simulink model "test_SimulinkMdl2_qLPVMPCbeta_UIO_testOL"  (R2019b)
settings: Solver=FixedStepAuto  StartTime=0.0  StopTime=400  FixedStep=DT  RelTol=1e-3
values from neighbouring files (symbols this model uses):
  beta = [-0.13962634015954636; -0.1361356816555577; -0.13264502315156904;          -0.12915436464758037; -0.12566370614359171; -0.12217304763960307;          -0.11868238913561441; -0.11519173063162574; -0.11170107212763709;          -0.10821041362364842; -0.10471975511965977; -0.10122909661567112;          -0.097738438111682452; -0.094247779607693788; -0.09075712110370511;          -0.087266462599716474;  ...(+3598 chars)    [MdlMFile.m]
  Cq = saveVarsMat.Cq    [MdlMFile.m]
  Ct = saveVarsMat.Ct    [MdlMFile.m]
  DT = 0.008    [LUTMFile.m]    (also in UIOLinestTr.m; exUIO_WECS.m; getFictInputMatricesOrd3M.m; initWorkspace.m)
  lambda = [0; 0.1; 0.2; 0.30000000000000004; 0.4; 0.5; 0.60000000000000009;            0.70000000000000007; 0.8; 0.9; 1; 1.1; 1.2000000000000002; 1.3;            1.4000000000000001; 1.5; 1.6; 1.7000000000000002; 1.8; 1.9000000000000001;            2; 2.1; 2.2; 2.3000000000000003; 2.4000000000000004; 2.5; 2.6;            2.7; 2.8000000000000003; 2.9000000000000004; 3; 3.1; 3.2; 3.3000000000000003;            ...(+1285 chars)    [MdlMFile.m]    (also in exLQR_hamiltonian.m = -10; koopmanKhalil.m = 1)
  Lin_points = 0.74811652133345019 0.78122947334555715 0.82586806925039735 0.88042797952230989 0.94564154658981237 1.06231329175348 1.1780905557148451 1.2402773842094346 1.254474305465946 1.2544764615597244 1.2544775037226534 1.2544778841663968 1.2544780221694662 1.2544779823335293 1.254477987181289 1.2544781738200332 1.254478189259095 1.2544780953600987 1.2544781548505395 1.2544783366942183 1.2544785605869417 1    [DD_test.sldd]    (also in LinPointsMFile.m = struct)
  rho = 1.2250    (= 1.225)    [ABqL_WT_est_matlab.m]    (also in MdlMFile.m; UIOLinestTr.m; getFictInputMatricesOrd3M.m; testTorqueFromomegaNonLin.m)
  sysEst = c2d(ss(F,[T*B,K],eye(nx),[zeros(size(T*B)),H]),DT,'zoh')    [exUIO_WECS.m]
  Vbar = rhoP(3)    [ABqL_WT_est_matlab.m]    (also in checkOPSimulink.m = Lin_points.V(index); createLinearModels.m = Lin.V(index); getFictInputMatricesOrd3M.m = wind - zetadot*rb - ytdot)
  wecs = 3.0    [DD_test.sldd]    (also in MdlMFile.m = struct)
undefined symbols (not defined in the file or in its folder): Rotor_Lambda
settings Model: ExtModeTrigMode=oneshot  ExtModeArmWhenConnect=off  Creator=Hazim Namik  LastModifiedBy=ditt_aj
settings DataIOCC: LimitDataPoints=on  SaveFormat=Array  ReturnWorkspaceOutputs=off
settings OptimizationCC: BlockReduction=off  BooleanDataType=off  LifeSpan=inf
settings DebuggingCC: SaveWithParameterizedLinksMsg=none  UnderspecifiedInitializationDetection=Classic  MergeDetectMultiDrivingBlocksExec=none  SignalResolutionControl=TryResolveAllWithWarning  SFUnexpectedBacktrackingDiag=warning  SFNoUnconditionalDefaultTransitionDiag=warning  SFExecutionAtInitializationDiag=none  ArithmeticOperatorsInVariantConditions=warning
settings HardwareCC: ProdBitPerPointer=32  ProdBitPerSizeT=32  ProdBitPerPtrDiffT=32  ProdLargestAtomicFloat=None  ProdIntDivRoundTo=Undefined  ProdEndianess=Unspecified  ProdWordSize=32  ProdHWDeviceType=32-bit Generic  TargetUnknown=on
settings ModelReferenceCC: PropagateSignalLabelsOutOfModel=off
settings SFSimCC: SimUseLocalCustomCode=off  CustomCodeUndefinedFunction=UseInterfaceOnly
settings RTWCC: RTWUseLocalCustomCode=off
settings CodeAppCC: StateflowObjectComments=on
settings GRTTargetCC: TargetLangStandard=C89/C90 (ANSI)  GeneratePreprocessorConditionals=Disable all
settings ConfigComp: CovMetricSettings=dw  CovHtmlReporting=on  CovSaveCumulativeToWorkspaceVar=on  CovSaveSingleToWorkspaceVar=on  CovExternalEMLEnable=off

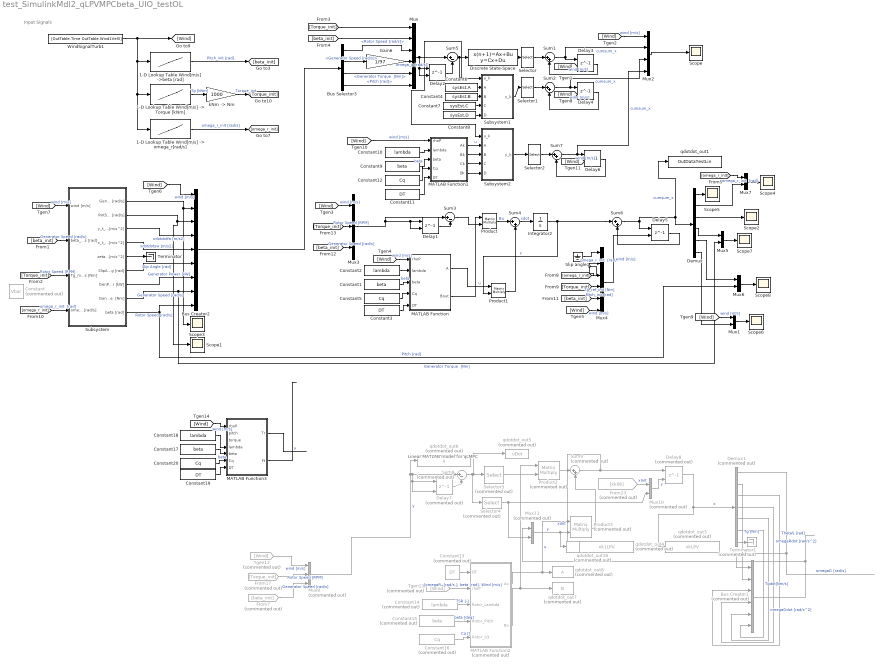
== system test_SimulinkMdl2_qLPVMPCbeta_UIO_testOL ==
  note: Input Signals
  note: Linear MATLAB model for qLMPC
  "1-D Lookup Table Wind[m/s] -> Torque [kNm]" : Lookup_n-D  NumberOfTableDimensions=1  BreakpointsForDimension1=Lin_points.V  BreakpointsForDimension2=Rotor_Lambda  Table=Lin_points.Torque  InternalRulePriority=Speed  RndMeth=Simplest  InputSameDT=on
  "1-D Lookup Table Wind[m/s] -> omega_r[rad/s]" : Lookup_n-D  NumberOfTableDimensions=1  BreakpointsForDimension1=Lin_points.V  BreakpointsForDimension2=Rotor_Lambda  Table=Lin_points.RSpeed  InternalRulePriority=Speed  RndMeth=Simplest  InputSameDT=on
  1-D Lookup Table Wind[m/s] ->beta [rad] : Lookup_n-D  NumberOfTableDimensions=1  BreakpointsForDimension1=Lin_points.V  BreakpointsForDimension2=Rotor_Lambda  Table=Lin_points.Pitch  InternalRulePriority=Speed  RndMeth=Simplest  InputSameDT=on
  Bus Creator1 : BusCreator  Commented=on  Inputs=6
  Bus Creator2 : BusCreator  Inputs=9
  Bus Selector3 : BusSelector  OutputSignals="Rotor Speed [rad/s],Generator Speed [rad/s],Generator Torque  [Nm],Pitch [rad]"
  Constant : Constant  Commented=on  Value=Vbar
  Constant1 : Constant  Value=beta
  Constant10 : Constant  Value=lambda
  Constant11 : Constant  Value=DT
  Constant12 : Constant  Value=Cq
  Constant13 : Constant  Commented=on  Value=DT
  Constant14 : Constant  Commented=on  Value=lambda
  Constant15 : Constant  Commented=on  Value=beta
  Constant16 : Constant  Commented=on  Value=Cq
  Constant17 : Constant  Value=beta
  Constant18 : Constant  Value=lambda
  Constant19 : Constant  Value=DT
  Constant2 : Constant  Value=lambda
  Constant20 : Constant  Value=Cq
  Constant3 : Constant  Value=DT
  Constant4 : Constant  Value=sysEst.B
  Constant5 : Constant  Value=Cq
  Constant6 : Constant  Value=sysEst.A
  Constant7 : Constant  Value=sysEst.C
  Constant8 : Constant  Value=sysEst.D
  Constant9 : Constant  Value=beta
  Delay{1..6} (6 alike) : Delay  DelayLength=1  InitialConditionSource=Input port  InitialCondition=0
      settings: InputPortMap=u0,p4
  Delay7 : Delay  Commented=on  DelayLength=1  InitialConditionSource=Input port  InitialCondition=[0, Lin_points.Torque(1)]
      settings: InputPortMap=u0,p4
  Delay8 : Delay  Commented=on  DelayLength=1  InitialConditionSource=Input port
      settings: InputPortMap=u0,p4
  Demux : Demux  Outputs=6
  Demux1 : Demux  Commented=on  Outputs=7
  Discrete State-Space : DiscreteStateSpace  A=sysEst.A  B=sysEst.B  C=sysEst.C  D=sysEst.D  SampleTime=DT
  From17 : From  Commented=on  GotoTag=Torque_init
      settings: CloseFcn=tagdialog Close
  From23 : From  Commented=on  GotoTag=xk06
      settings: CloseFcn=tagdialog Close
  From7 : From  Commented=on  GotoTag=beta_init
      settings: CloseFcn=tagdialog Close
  Gain6 : Gain  Gain=1/97
  Integrator2 : Integrator
  MATLAB Function : MATLAB Function  TreatAsAtomicUnit=on
  MATLAB Function1 : MATLAB Function  TreatAsAtomicUnit=on
  MATLAB Function2 : MATLAB Function  Commented=on  TreatAsAtomicUnit=on
  MATLAB Function3 : MATLAB Function  TreatAsAtomicUnit=on
  Mux : Mux  Inputs=6
  Mux{1,5..7} (4 alike) : Mux  Inputs=2
  Mux10 : Mux  Commented=on  Inputs=2
  Mux11 : Mux  Commented=on  Inputs=2
  Mux2 : Mux
  Mux3 : Mux  Inputs=3
  Mux4 : Mux  Inputs=6
  Mux8 : Mux  Commented=on  Inputs=3
  Product : Product  Multiplication=Matrix(*)
  Product1 : Product  Multiplication=Matrix(*)
  Product2 : Product  Commented=on  Multiplication=Matrix(*)  RndMeth=Zero
  Product3 : Product  Commented=on  Multiplication=Matrix(*)  RndMeth=Zero
  Scope{,1..8} (9 alike) : Scope
  Selector : Selector  InputPortWidth=size(sysEst.C,1)  IndexOptions=Index vector (dialog)  Indices=size(sysEst.C,1)  OutputSizes=1
  Selector1 : Selector  InputPortWidth=size(sysEst.C,1)  IndexOptions=Index vector (dialog)  Indices=size(sysEst.C,1)  OutputSizes=1
  Selector2 : Selector  InputPortWidth=size(sysEst.C,1)  IndexOptions=Index vector (dialog)  Indices=size(sysEst.C,1)  OutputSizes=1
  Selector3 : Selector  Commented=on  InputPortWidth=3  IndexOptions=Index vector (dialog)  Indices=[2 3]  OutputSizes=1
  Selector4 : Selector  Commented=on  InputPortWidth=3  IndexOptions=Index vector (dialog)  Indices=1  OutputSizes=1
  Slip angle1 : Ground
  Subsystem : Subsystem
  Subsystem1 : Subsystem
  Subsystem2 : Subsystem
  Sum{1..2,4,6..7} (5 alike) : Sum  Inputs=|++
  Sum3 : Sum  Inputs=|+-
  Sum5 : Sum  Inputs=|+-
  Sum8 : Sum  Commented=on  Inputs=|+-
  Sum9 : Sum  Commented=on  Inputs=|++
  Terminator : Terminator
  Terminator1 : Terminator  Commented=on
  Tgen12 : From  Commented=on  GotoTag=Wind
      settings: CloseFcn=tagdialog Close
  Tgen13 : From  Commented=on  GotoTag=Wind
      settings: CloseFcn=tagdialog Close
  WindSignalTurb1 : FromWorkspace  VariableName=[OutTable.Time OutTable.Wind1VelX]  SampleTime=DT  OutputAfterFinalValue=Holding final value
  "kNm -> Nm" : Gain  Gain=1000
  qdotdot_out1 : ToWorkspace  VariableName=OutDataTestLin  SampleTime=-1
  qdotdot_out19 : ToWorkspace  Commented=on  VariableName=xkLPV1  SampleTime=-1
  qdotdot_out3 : ToWorkspace  Commented=on  VariableName=xkLPV  SampleTime=-1
  qdotdot_out4 : ToWorkspace  Commented=on  VariableName=xk1LPV  SampleTime=-1
  qdotdot_out5 : ToWorkspace  Commented=on  VariableName=uDot  SampleTime=-1
  qdotdot_out6 : ToWorkspace  Commented=on  VariableName=u  SampleTime=-1
  qdotdot_out7 : ToWorkspace  Commented=on  VariableName=B  SampleTime=-1
  qdotdot_out8 : ToWorkspace  Commented=on  VariableName=A  SampleTime=-1
  wires:
  Subsystem/7(GenPwr [kW]) -> Bus Creator2/7  "Generator Power [kW]"
  WindSignalTurb1/1 -> [Wind], "1-D Lookup Table Wind[m/s] -> omega_r[rad/s]"/1, "1-D Lookup Table Wind[m/s] -> Torque [kNm]"/1, 1-D Lookup Table Wind[m/s] ->beta [rad]/1
  Subsystem/3(y_t_dotdot [m/s^2]) -> Bus Creator2/4  "xdotdotfa [m/s2]"
  Subsystem/6(SlipAng [rad]) -> Bus Creator2/6  "Slip Angle [rad]"
  "kNm -> Nm"/1 -> [Torque_init]  "Torque_init"
  Bus Creator2/1 -> Bus Selector3/1
  Subsystem/2(" RotSpeed [rad/s]") -> Scope1/1, Bus Creator2/3  "Rotor Speed [rad/s]"
  [Torque_init] -> Subsystem/3(Tg_meas [Nm])  "Rotor Speed [RPM]"
  [Wind] -> Bus Creator2/1  "wind [m/s]"
  Subsystem/4(x_t_dotdot [m/s^2]) -> Bus Creator2/5  "xdotdotsw [m/s2]"
  Subsystem/1("GenSpeed [rad/s] ") -> Scope3/1, Bus Creator2/2  "Generator Speed [rad/s]"
  "1-D Lookup Table Wind[m/s] -> omega_r[rad/s]"/1 -> [omega_r_init]  "omega_r_init [rad/s]"
  [Wind] -> Subsystem/1(wind [m/s])  "wind [m/s]"
  1-D Lookup Table Wind[m/s] ->beta [rad]/1 -> [beta_init]  "Pitch_init [rad]"
  "1-D Lookup Table Wind[m/s] -> Torque [kNm]"/1 -> "kNm -> Nm"/1  "Tg [kNm]"
  Subsystem/9(beta [rad]) -> Bus Creator2/9, Mux6/2  "Pitch [rad]"
  Subsystem/8("GenTorque  [Nm]  ") -> Mux5/2, Bus Creator2/8  "Generator Torque  [Nm]"
  Subsystem/5(zeta_dotdot [m/s^2]) -> Terminator/1
  [beta_init] -> Subsystem/2(beta_meas [rad])  "Generator Speed [rad/s]"
  [omega_r_init] -> Subsystem/4(omega_init [rad/s])  "omega_r_init  [rad]"
  Bus Selector3/1 -> Mux/3  "<Rotor Speed [rad/s]>"
  Bus Selector3/2 -> Gain6/1  "<Generator Speed [rad/s]>"
  Discrete State-Space/1 -> Selector/1
  Mux2/1 -> Scope/1
  [Wind] -> Mux2/1  "wind [m/s]"
  Subsystem1/1(y_k) -> Selector1/1
  [Torque_init] -> Mux/1
  [beta_init] -> Mux/2
  Bus Selector3/4 -> Mux/6  "<Pitch [rad]>"
  Bus Selector3/3 -> Mux/5  "<Generator Torque  [Nm]>"
  Gain6/1 -> Mux/4  "omega_g [rad/s]]"
  Constant2/1 -> MATLAB Function/2(lambda)
  Constant5/1 -> MATLAB Function/4(Cq)
  Constant1/1 -> MATLAB Function/3(beta)  "beta"
  Product/1 -> Sum4/1  "Bu"
  Integrator2/1 -> Sum6/1, Product1/2  "x"
  Sum4/1 -> Integrator2/1  "xdot"
  MATLAB Function/1(A) -> Product1/1  "u"
  MATLAB Function/2(Bout) -> Product/1
  Product1/1 -> Sum4/2
  Demux/3 -> Scope2/1
  Slip angle1/1 -> Mux4/1
  [beta_init] -> Mux4/5  "Pitch_init [rad]"
  [omega_r_init] -> Mux4/2, Mux4/3  "omega_r_init  [rad]"
  [Torque_init] -> Mux4/4  "Tg_ref_init [Nm]"
  Demux/1 -> Scope5/1
  Demux/4 -> Mux5/1
  Mux5/1 -> Scope7/1
  Mux6/1 -> Scope8/1
  Demux/5 -> Mux6/1
  [Wind] -> Mux3/1  "wind [m/s]"
  [beta_init] -> Mux3/3  "Generator Speed [rad/s]"
  [Torque_init] -> Mux3/2  "Rotor Speed [RPM]"
  Mux7/1 -> Scope4/1
  Mux3/1 -> Delay1/2, Delay1/1, Sum3/1
  Delay1/1 -> Sum3/2
  Sum3/1 -> Product/2
  [Wind] -> MATLAB Function/1(rhoP)  "wind [m/s]"
  Constant3/1 -> MATLAB Function/5(DT)
  [Wind] -> Mux4/6  "wind [m/s]"
  Sum1/1 -> Delay3/1, Mux2/2  "cumsum_x"
  Delay3/1 -> Sum1/2
  [Wind] -> Delay3/2  "wind [m/s]"
  Selector/1 -> Sum1/1
  Sum2/1 -> Mux2/3, Delay4/1  "cumsum_x"
  [Wind] -> Delay4/2  "wind [m/s]"
  Delay4/1 -> Sum2/2
  Selector1/1 -> Sum2/1
  Mux/1 -> Delay2/1, Delay2/2, Sum5/1
  Delay2/1 -> Sum5/2
  Sum5/1 -> Subsystem2/1(u_k), Subsystem1/1(u_k), Discrete State-Space/1
  Mux4/1 -> Delay5/2  "wind [m/s]"
  Delay5/1 -> Sum6/2
  Sum6/1 -> qdotdot_out1/1, Demux/1, Delay5/1  "cumsum_x"
  Mux1/1 -> Scope6/1
  Demux/6 -> Mux1/2
  [Wind] -> Mux1/1  "wind [m/s]"
  Constant6/1 -> Subsystem1/2(A)
  Constant4/1 -> Subsystem1/3(B)
  Constant7/1 -> Subsystem1/4(C)
  Constant8/1 -> Subsystem1/5(D)
  [Wind] -> MATLAB Function1/1(rhoP)  "wind [m/s]"
  Constant10/1 -> MATLAB Function1/2(lambda)
  Constant12/1 -> MATLAB Function1/4(Cq)
  Constant9/1 -> MATLAB Function1/3(beta)  "beta"
  Constant11/1 -> MATLAB Function1/5(DT)
  MATLAB Function1/1(Ak) -> Subsystem2/2(A)  "u"
  MATLAB Function1/2(Bk) -> Subsystem2/3(B)
  MATLAB Function1/3(Ck) -> Subsystem2/4(C)
  MATLAB Function1/4(Dk) -> Subsystem2/5(D)
  Selector2/1 -> Sum7/1
  [Wind] -> Delay6/2  "wind [m/s]"
  Delay6/1 -> Sum7/2
  Sum7/1 -> Mux2/4, Delay6/1  "cumsum_x"
  Subsystem2/1(y_k) -> Selector2/1
  Demux/2 -> Mux7/2
  [omega_r_init] -> Mux7/1  "omega_r_init  [rad]"
  Mux8/1 -> qdotdot_out6/1, Delay7/1, Delay7/2, Sum8/1  "y"
  Selector4/1 -> Mux11/2, Mux10/2
  Selector3/1 -> Product2/2
  MATLAB Function2/2(Bv) -> qdotdot_out7/1, Product2/1
  Demux1/2 -> Bus Creator1/2  "Tg [Nm]"
  Sum9/1 -> Delay8/1, qdotdot_out4/1  "xdot"
  MATLAB Function2/1(Av) -> Product3/1, qdotdot_out8/1  "u"
  Sum8/1 -> Selector4/1, Selector3/1, qdotdot_out5/1
  Delay8/1 -> Demux1/1, qdotdot_out3/1  "x"
  Tgen13/1 -> MATLAB Function2/2(rhoP)  "[omegaR  [rad/s,], beta [rad], Wind [m/s]"
  Mux11/1 -> qdotdot_out19/1, Product3/2  "y"
  Bus Creator1/1 -> Mux11/1
  Demux1/5 -> Bus Creator1/5  "omegaGdot [rad/s^2]"
  Demux1/4 -> Bus Creator1/4  "omegaRdot [rad/s^2]"
  Demux1/3 -> Bus Creator1/3  "ThetaS [rad]"
  Demux1/7 -> Terminator1/1
  Delay7/1 -> Sum8/2
  Constant15/1 -> MATLAB Function2/4(Rotor_Pitch)  "beta [deg]"
  Demux1/1 -> Bus Creator1/1  "omegaG [rad/s]"
  Demux1/6 -> Bus Creator1/6  "Tgdot[Nm/s]"
  Mux10/1 -> Delay8/2  "y"
  Constant13/1 -> MATLAB Function2/1(DT)
  Product2/1 -> Sum9/1
  Constant16/1 -> MATLAB Function2/5(Rotor_cQ)  "Cq []"
  Constant14/1 -> MATLAB Function2/3(Rotor_Lambda)  "TSR [-]"
  From23/1 -> Mux10/1  "xInit"
  Product3/1 -> Sum9/2
  Tgen12/1 -> Mux8/1  "wind [m/s]"
  From17/1 -> Mux8/2  "Rotor Speed [RPM]"
  From7/1 -> Mux8/3  "Generator Speed [rad/s]"
  Constant19/1 -> MATLAB Function3/7(DT)
  MATLAB Function3/2(Ft) -> ?
  Constant17/1 -> MATLAB Function3/5(beta)  "beta"
  MATLAB Function3/1(Tr) -> ?  "u"
  Constant20/1 -> MATLAB Function3/6(Cq)
  [Wind] -> MATLAB Function3/1(rhoP)  "wind [m/s]"
  Constant18/1 -> MATLAB Function3/4(lambda)

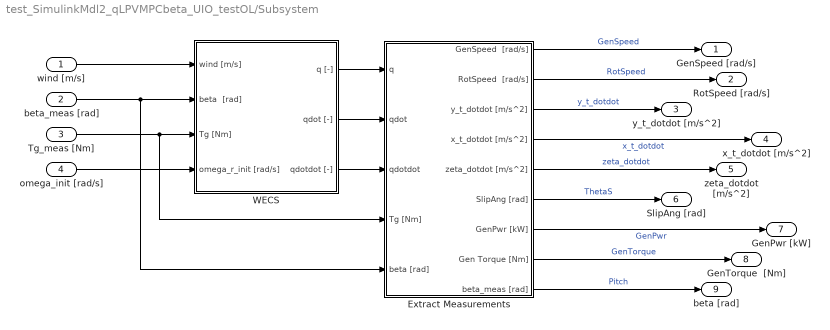
== system test_SimulinkMdl2_qLPVMPCbeta_UIO_testOL/Subsystem ==
  wind [m/s] : Inport
  beta_meas [rad] : Inport  Port=2
  Tg_meas [Nm] : Inport  Port=3
  omega_init [rad/s] : Inport  Port=4
  Extract Measurements : Subsystem
  WECS : Subsystem
  "GenSpeed [rad/s] " : Outport  VectorParamsAs1DForOutWhenUnconnected=off
  " RotSpeed [rad/s]" : Outport  Port=2  VectorParamsAs1DForOutWhenUnconnected=off
  y_t_dotdot [m/s^2] : Outport  Port=3  VectorParamsAs1DForOutWhenUnconnected=off
  x_t_dotdot [m/s^2] : Outport  Port=4  VectorParamsAs1DForOutWhenUnconnected=off
  zeta_dotdot [m/s^2] : Outport  Port=5  VectorParamsAs1DForOutWhenUnconnected=off
  SlipAng [rad] : Outport  Port=6  VectorParamsAs1DForOutWhenUnconnected=off
  GenPwr [kW] : Outport  Port=7  VectorParamsAs1DForOutWhenUnconnected=off
  "GenTorque  [Nm]  " : Outport  Port=8  VectorParamsAs1DForOutWhenUnconnected=off
  beta [rad] : Outport  Port=9  VectorParamsAs1DForOutWhenUnconnected=off
  wires:
  omega_init [rad/s]/1 -> WECS/4(omega_r_init [rad/s])
  beta_meas [rad]/1 -> WECS/2(beta  [rad]), Extract Measurements/5(beta [rad])
  Extract Measurements/3(y_t_dotdot [m/s^2]) -> y_t_dotdot [m/s^2]/1  "y_t_dotdot"
  wind [m/s]/1 -> WECS/1(wind [m/s])
  Extract Measurements/8("Gen Torque [Nm]  ") -> "GenTorque  [Nm]  "/1  "GenTorque"
  Extract Measurements/4(x_t_dotdot [m/s^2]) -> x_t_dotdot [m/s^2]/1  "x_t_dotdot"
  WECS/1(q [-]) -> Extract Measurements/1(q)
  Tg_meas [Nm]/1 -> WECS/3(Tg [Nm]), Extract Measurements/4(Tg [Nm])
  Extract Measurements/5(zeta_dotdot [m/s^2]) -> zeta_dotdot [m/s^2]/1  "zeta_dotdot"
  Extract Measurements/2(RotSpeed  [rad/s]) -> " RotSpeed [rad/s]"/1  "RotSpeed"
  WECS/2(qdot [-]) -> Extract Measurements/2(qdot)
  Extract Measurements/1(GenSpeed  [rad/s]) -> "GenSpeed [rad/s] "/1  "GenSpeed"
  Extract Measurements/9(beta_meas [rad]) -> beta [rad]/1  "Pitch"
  Extract Measurements/6(SlipAng [rad]) -> SlipAng [rad]/1  "ThetaS"
  WECS/3(qdotdot [-]) -> Extract Measurements/3(qdotdot)
  Extract Measurements/7(GenPwr [kW]) -> GenPwr [kW]/1  "GenPwr"

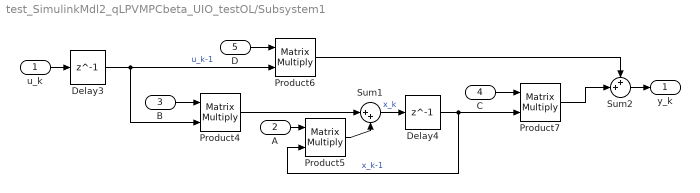
== system test_SimulinkMdl2_qLPVMPCbeta_UIO_testOL/Subsystem1 ==
  u_k : Inport
  A : Inport  Port=2
  B : Inport  Port=3
  C : Inport  Port=4
  D : Inport  Port=5
  Delay3 : Delay  DelayLength=1
  Delay4 : Delay  DelayLength=1
  Product{4..7} (4 alike) : Product  Multiplication=Matrix(*)
  Sum1 : Sum  Inputs=|++
  Sum2 : Sum  Inputs=++|
  y_k : Outport
  wires:
  Delay4/1 -> Product5/2, Product7/2  "x_k-1"
  u_k/1 -> Delay3/1
  Product7/1 -> Sum2/2
  C/1 -> Product7/1
  Product6/1 -> Sum2/1
  Delay3/1 -> Product4/2, Product6/2  "u_k-1"
  Product5/1 -> Sum1/2
  D/1 -> Product6/1
  Product4/1 -> Sum1/1
  A/1 -> Product5/1
  Sum1/1 -> Delay4/1  "x_k"
  B/1 -> Product4/1
  Sum2/1 -> y_k/1

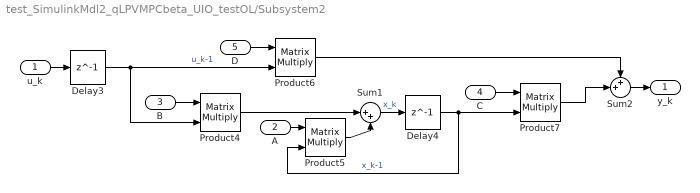
== system test_SimulinkMdl2_qLPVMPCbeta_UIO_testOL/Subsystem2 ==
  u_k : Inport
  A : Inport  Port=2
  B : Inport  Port=3
  C : Inport  Port=4
  D : Inport  Port=5
  Delay3 : Delay  DelayLength=1
  Delay4 : Delay  DelayLength=1
  Product{4..7} (4 alike) : Product  Multiplication=Matrix(*)
  Sum1 : Sum  Inputs=|++
  Sum2 : Sum  Inputs=++|
  y_k : Outport
  wires:
  Delay4/1 -> Product5/2, Product7/2  "x_k-1"
  u_k/1 -> Delay3/1
  Product7/1 -> Sum2/2
  C/1 -> Product7/1
  Product6/1 -> Sum2/1
  Delay3/1 -> Product4/2, Product6/2  "u_k-1"
  Product5/1 -> Sum1/2
  D/1 -> Product6/1
  Product4/1 -> Sum1/1
  A/1 -> Product5/1
  Sum1/1 -> Delay4/1  "x_k"
  B/1 -> Product4/1
  Sum2/1 -> y_k/1

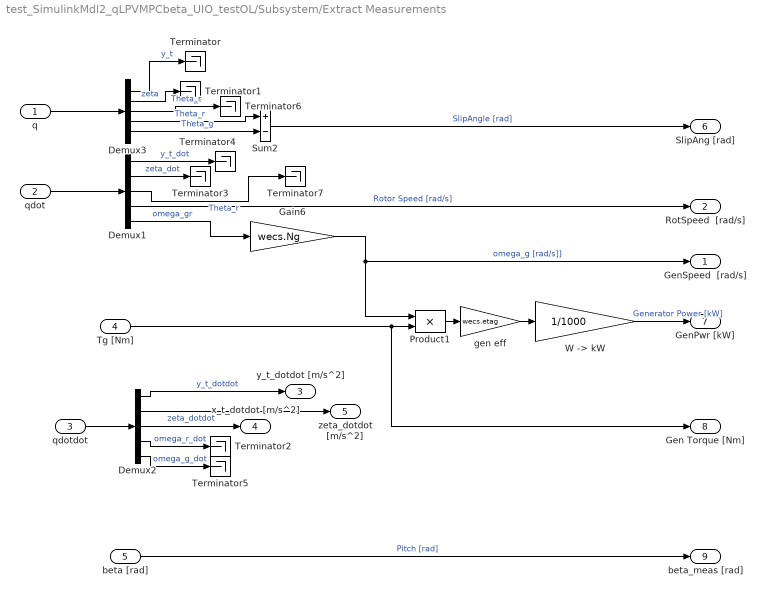
== system test_SimulinkMdl2_qLPVMPCbeta_UIO_testOL/Subsystem/Extract Measurements ==
  q : Inport
  qdot : Inport  Port=2
  qdotdot : Inport  Port=3
  Tg [Nm] : Inport  Port=4
  beta [rad] : Inport  Port=5
  Demux1 : Demux  Outputs=5
  Demux2 : Demux  Outputs=5
  Demux3 : Demux  Outputs=5
  Gain6 : Gain  Gain=wecs.Ng
  Product1 : Product  RndMeth=Zero
  Sum2 : Sum  Inputs=+-
  Terminator{,1..7} (8 alike) : Terminator
  "W -> kW" : Gain  Gain=1/1000
  gen eff : Gain  Gain=wecs.etag
  GenSpeed  [rad/s] : Outport  VectorParamsAs1DForOutWhenUnconnected=off
  RotSpeed  [rad/s] : Outport  Port=2  VectorParamsAs1DForOutWhenUnconnected=off
  y_t_dotdot [m/s^2] : Outport  Port=3  VectorParamsAs1DForOutWhenUnconnected=off
  x_t_dotdot [m/s^2] : Outport  Port=4  VectorParamsAs1DForOutWhenUnconnected=off
  zeta_dotdot [m/s^2] : Outport  Port=5  VectorParamsAs1DForOutWhenUnconnected=off
  SlipAng [rad] : Outport  Port=6  VectorParamsAs1DForOutWhenUnconnected=off
  GenPwr [kW] : Outport  Port=7  VectorParamsAs1DForOutWhenUnconnected=off
  "Gen Torque [Nm]  " : Outport  Port=8  VectorParamsAs1DForOutWhenUnconnected=off
  beta_meas [rad] : Outport  Port=9  VectorParamsAs1DForOutWhenUnconnected=off
  wires:
  Demux1/2 -> Terminator3/1  "zeta_dot"
  Demux2/1 -> y_t_dotdot [m/s^2]/1  "y_t_dotdot"
  Gain6/1 -> GenSpeed  [rad/s]/1, Product1/1  "omega_g [rad/s]]"
  Demux1/1 -> Terminator4/1  "y_t_dot"
  qdot/1 -> Demux1/1
  Demux3/4 -> Sum2/1  "Theta_r"
  Demux3/5 -> Sum2/2  "Theta_g"
  Demux2/5 -> Terminator5/1  "omega_g_dot"
  Tg [Nm]/1 -> "Gen Torque [Nm]  "/1, Product1/2
  Demux2/4 -> Terminator2/1  "omega_r_dot"
  Sum2/1 -> SlipAng [rad]/1  "SlipAngle [rad]"
  Demux1/5 -> Gain6/1  "omega_gr"
  Product1/1 -> gen eff/1
  Demux3/2 -> Terminator1/1  "zeta"
  Demux2/2 -> zeta_dotdot [m/s^2]/1  "zeta_dotdot"
  Demux3/1 -> Terminator/1  "y_t"
  gen eff/1 -> "W -> kW"/1
  "W -> kW"/1 -> GenPwr [kW]/1  "Generator Power [kW]"
  q/1 -> Demux3/1
  qdotdot/1 -> Demux2/1
  Demux1/4 -> RotSpeed  [rad/s]/1  "Rotor Speed [rad/s]"
  beta [rad]/1 -> beta_meas [rad]/1  "Pitch [rad]"
  Demux2/3 -> x_t_dotdot [m/s^2]/1
  Demux3/3 -> Terminator6/1  "Theta_r"
  Demux1/3 -> Terminator7/1  "Theta_r"

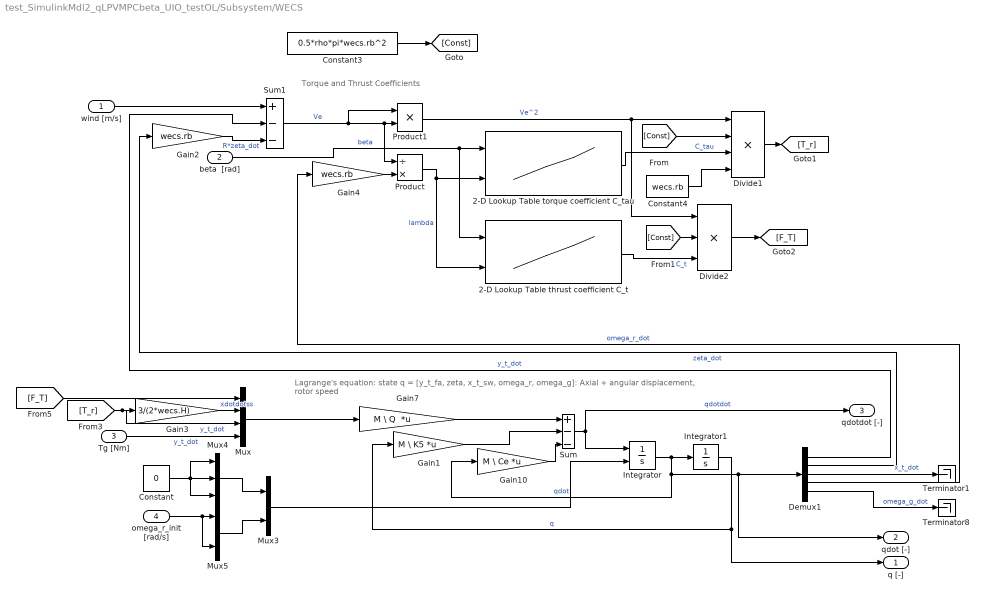
== system test_SimulinkMdl2_qLPVMPCbeta_UIO_testOL/Subsystem/WECS ==
  note: Torque and Thrust Coefficients
  note: Lagrange's equation: state q = [y_t_fa, zeta, x_t_sw, omega_r, omega_g]:
      |  Axial  + angular displacement, rotor speed
  wind [m/s] : Inport
  beta  [rad] : Inport  Port=2
  Tg [Nm] : Inport  Port=3
  omega_r_init [rad/s] : Inport  Port=4
  2-D Lookup Table thrust coefficient C_t : Lookup_n-D  BreakpointsForDimension1=beta  BreakpointsForDimension2=lambda  Table=Ct  InterpMethod=Cubic spline  InternalRulePriority=Speed  RndMeth=Simplest  InputSameDT=on
  2-D Lookup Table torque coefficient C_tau : Lookup_n-D  BreakpointsForDimension1=beta  BreakpointsForDimension2=lambda  Table=Cq  InterpMethod=Cubic spline  InternalRulePriority=Speed  RndMeth=Simplest  InputSameDT=on
  Constant : Constant  Value=0
  Constant3 : Constant  Value=0.5*rho*pi*wecs.rb^2
  Constant4 : Constant  Value=wecs.rb
  Demux1 : Demux  Outputs=5
  Divide1 : Product  Inputs=****
  Divide2 : Product  Inputs=***
  Gain1 : Gain  Gain=M \ K5  Multiplication=Matrix(K*u)
  Gain10 : Gain  Gain=M \ Ce  Multiplication=Matrix(K*u)
  Gain2 : Gain  Gain=wecs.rb
  Gain3 : Gain  Gain=3/(2*wecs.H)
  Gain4 : Gain  Gain=wecs.rb
  Gain7 : Gain  Gain=M \ Q  Multiplication=Matrix(K*u)
  Integrator : Integrator  InitialConditionSource=external  InitialCondition=[0,0,0.75, 0.75]
  Integrator1 : Integrator  InitialCondition=[0,0,0,0,0]
  Mux : Mux
  Mux3 : Mux  Inputs=2
  Mux4 : Mux  Inputs=3
  Mux5 : Mux  Inputs=2
  Product : Product  Inputs=/*
  Product1 : Product  Inputs=**
  Sum : Sum  Inputs=+--
  Sum1 : Sum  Inputs=+--
  Terminator1 : Terminator
  Terminator8 : Terminator
  q [-] : Outport  VectorParamsAs1DForOutWhenUnconnected=off
  qdot [-] : Outport  Port=2  VectorParamsAs1DForOutWhenUnconnected=off
  qdotdot [-] : Outport  Port=3  VectorParamsAs1DForOutWhenUnconnected=off
  wires:
  Constant4/1 -> Divide1/4
  Sum1/1 -> Product1/1, Product1/2, Product/1  "Ve"
  wind [m/s]/1 -> Sum1/1
  Gain4/1 -> Product/2
  Divide2/1 -> [F_T]
  2-D Lookup Table thrust coefficient C_t/1 -> Divide2/3  "C_t"
  Divide1/1 -> [T_r]
  [Const] -> Divide1/2
  [Const] -> Divide2/2
  2-D Lookup Table torque coefficient C_tau/1 -> Divide1/3  "C_tau"
  Gain1/1 -> Sum/2
  Gain7/1 -> Sum/1
  Mux/1 -> Gain7/1
  Integrator1/1 -> Gain1/1, q [-]/1  "q"
  [F_T] -> Mux/1
  Demux1/1 -> Sum1/2  "y_t_dot"
  Demux1/2 -> Gain2/1  "zeta_dot"
  Demux1/4 -> Gain4/1  "omega_r_dot"
  Gain2/1 -> Sum1/3  "R*zeta_dot"
  beta  [rad]/1 -> 2-D Lookup Table thrust coefficient C_t/1, 2-D Lookup Table torque coefficient C_tau/1  "beta"
  Product/1 -> 2-D Lookup Table thrust coefficient C_t/2, 2-D Lookup Table torque coefficient C_tau/2  "lambda"
  Product1/1 -> Divide1/1, Divide2/1  "Ve^2"
  Integrator/1 -> Gain10/1, Demux1/1, qdot [-]/1, Integrator1/1  "qdot"
  Gain10/1 -> Sum/3
  Constant3/1 -> [Const]
  [T_r] -> Mux/3, Gain3/1  "y_t_dot"
  Sum/1 -> Integrator/1, qdotdot [-]/1  "qdotdot"
  Mux4/1 -> Mux3/1
  Mux3/1 -> Integrator/2
  Constant/1 -> Mux4/3, Mux4/1, Mux4/2
  Mux5/1 -> Mux3/2
  omega_r_init [rad/s]/1 -> Mux5/2, Mux5/1
  Tg [Nm]/1 -> Mux/4  "y_t_dot"
  Demux1/3 -> Terminator1/1  "x_t_dot"
  Demux1/5 -> Terminator8/1  "omega_g_dot"
  Gain3/1 -> Mux/2  "xdotdotss"

== matlab function test_SimulinkMdl2_qLPVMPCbeta_UIO_testOL/MATLAB Function1 ==
  settings: updateMethod=DISCRETE
  data: rhoP input; lambda input; beta input; Cq input; Ak output; Bk output; DT input; Ck output; Dk output
function [Ak,Bk,Ck,Dk]  = ABqL_WT_est_m(rhoP,lambda,beta,Cq,DT)
% ABqL calculates system (A) and input (B) matrix for quasiLPV
% representation for ve
%
% Inputs: * Ts: Sampling time
%         * AwithV: Scheduling parameter vector: AwithV = V
%
% Outputs: * A: System matrix A(AwithV) at current estimated air speed AwithV, discretised with Ts
%          * B: Input matrix B(AwithV) at current AwithV, discretised with Ts

% Pablo S.G. Cisneros, Herbert Werner, ICS TUHH
% modified for WECS simulation: Antje Dittmer

persistent lambdaVec pitchVec CqVec Cqdlambda Cqdbeta

if isempty(lambdaVec)
    lambdaVec =  lambda;
    pitchVec = beta;
    CqVec = Cq;
    %% Compute gradients %%[Cpdlambda,Cpdbeta] = gradient(Cp,mean(diff(Xq(1,:))),mean(diff(Yq(:,1))));
    [Cqdlambda,Cqdbeta] = gradient(CqVec,mean(diff(lambda)),mean(diff(beta))); %dcQ/dbetaDeg * dbetaDeg/dbetaRad *betaRAd
end

%% Parameters
if length(rhoP) == 1
    Vbar = rhoP; % Vbar
    LUT_V = 4:25; % LUT table rows
    
    LUT_omega = ...%[0.4815, 0.6017,0.7217,0.8413,0.9603,1.0786,1.1949, repmat(1.2671,1,15)];
        [0.7458832277625318 0.77759738173519954 0.820732502042672 ...
        0.87379091011167287 0.93538972625666472 1.0429417531956238 ...
        1.1591854391157337 1.2371015764176956 1.2554479267196832 ...
        1.2547857982936621 1.2545286368009017 1.2546177195393646 ...
        1.2545376249695805 1.2545426663335242 1.2545426663335242 ...
        1.2545426663335242 1.2545426663335242 1.2545426663335242 ...
        1.2545426663335242 1.2545426663335242 1.2545426663335242 ...
        1.2545426663335242];
    
    LUT_beta =  [0 0 0 0 0 0 0 0 0.064193209888351435 0.11259119004615419 ...
        0.14929546421559495 0.18081611050661253 0.20926497731412011 ...
        0.23701571242082992 0.26197392072434883 0.28536133270107289 ...
        0.30770154712660031 0.32934362985133 0.35028758087526196 ...
        0.37035886727319672 0.38973202197033374 0.40858157789187255 ...
        ];
    
    
    % Get omegabar and beta
    omegabar = interp1(LUT_V,LUT_omega,Vbar,'pchip');
    beta_bar = interp1(LUT_V,LUT_beta,Vbar,'pchip');
    
elseif length(rhoP) == 3
    % rho = xdotk_1([1,3,4]); % Tg not included: [Omega [1/s], beta[rad], V [m/s]];
    Vbar = rhoP(3);
    omegabar = rhoP(1); % pass OmegaR OmegaG/Ng as approximation of omegaR
    beta_bar = rhoP(2);
    
else
    error('Unexpected length of scheduling parameter rho')
end

%% Physical and model constants
rho = 1.2250;
rb = 63; % m blade radius
Ng = 97; %Gearbox ratio
Jr = (115926 + 3 * 11.776e6) *1; %kg*m^2 Inertia of the rotor (Hub inertia + 3 blades
Jg = 534.116;% * Ng^2; %kg*m^2 Inertia of the generator (HSS)
Jgr = Jg * Ng^2; % Inertia of the generator in LSS
Ks = 867637000; %Nm/rad Stiffness of the transmission
Bs = 6215000;  %Nm/rad/sec        %Damping of the transmission
tau_g = 0.01; % for pitch actuator and airspeed

%% Lambda
Lambda_bar = omegabar*rb/Vbar;
dlambdadomega= rb/Vbar;
dlambdadV = - omegabar*rb/Vbar^2;

%% Grid points
Cqb = interp2(lambdaVec,pitchVec,Cq,Lambda_bar,beta_bar);
dCqdlambdab = interp2(lambdaVec,pitchVec,Cqdlambda,Lambda_bar,beta_bar);
dCqdbetab = interp2(lambdaVec,pitchVec,Cqdbeta,Lambda_bar,beta_bar);

%% Tr=0.5*pi*rb^3*Cq*v^2
dTrdomega = 0.5*rho*pi*rb^3*(dCqdlambdab*dlambdadomega)*Vbar^2;% br = dTr/domega
dTrdbeta = 0.5*rho*pi*rb^3*dCqdbetab*Vbar^2;% Krb = dTr/dbeta
dTrdV =  2*0.5*rho*pi*rb^3*Vbar*Cqb + ...
    0.5*rho*pi*rb^3*Vbar^2*dCqdlambdab*dlambdadV;

%% Create system matrix A:
% States: [Theta_s [rad], omega_r [rad/s], omega_gr [rad/s], T_g [Nm]]
% States for model xA = [y, xdot] with y = [Tg, beta]
% x = [ThetaS, OmegaR, OmegaG, Tg, beta,]
Atemp = [[0,1,-1,0] ;
    [-Ks/Jr, (-Bs + dTrdomega)/Jr, Bs/Jr,0];
    Ks/Jgr, Bs/Jgr, -Bs/Jgr, -Ng/Jgr;
    zeros(1,3), -1/tau_g];

%% Create input matrix B
% Input orig model: V [m/s], T_g_ref [Nm], beta [rad],
% -> vel model: Vdot [m/s^2]  , T_g_refDot [Nm/s]
% for beta: Vdot [m/s^2]  T_g_refDot [Nm/s] betaDot [rad/s],
Btemp = [zeros(1,3); dTrdV/Jr, 0 dTrdbeta/Jr; zeros(1,3);  0,  1/tau_g,0];

% With Beta
Aeval = [Atemp,Btemp(:,3); zeros(1, size(Atemp,2)), -1/tau_g];
Beval = [Btemp; zeros(1, size(Btemp,2))];
Beval(:,3) = 0;
Beval(end,3) = 1/tau_g;

%% Check rank
Bu = Beval(:,2:3);
Bd = Beval(:,1);
nxEval = size(Aeval,2);

% Also create an additional state for the disturbance
tau1 =  1/DT;
A =[[Aeval, zeros(nxEval,1)]; [zeros(1,nxEval),-tau1]];
E = [Bd;tau1]; %xd_dot = -xd + Ed
B = [Bu; zeros(1,2)];

%% Calculate observer matrices
Ceval = [zeros(nxEval-1,1),eye(nxEval-1)]; %
nyEval = size(Ceval,1);

C = [Ceval, zeros(nyEval,1)]; %[zeros(1,nx),1]];
H = E*inv((C*E)'*(C*E))*(C*E)'; %#ok<MINV,*NOPTS> display output, inv is fast enough
nx = size(A,1);
T = eye(nx)-H*C;
A1 = T*A;

% Pole placement with Q and R
Qe = [E,B]*[E,B]'; %
Re = C*C';
%K1 = lqr(A',C',Qe,Re)'; % lqr not supported in Simulink

Ham = [A', -C'* Re^(-1) * C; % Hamiltonion matrix -lambda to make it stabizable
    -Qe, -A]; 
[V,D] = eig(Ham); % Divide into stable and unstable eigenvalues
idxS = diag(D) < 0; % get stable eigenvalues
Vs = V(:,idxS);% get eigenvectors of stable eigenvalues
n11 = sum(idxS);
P = Vs(n11+1:end,:)/(Vs(1:n11,:));
K1 = real(Re^(-1) * C * P)';

% Calculate F and K
F = A1 - K1*C; %T*A -K1*C
K = K1 + F*H;
T = eye(size(H*C)) - H*C;

% Sys with no ctrl input: xdot = Ax + Ed, y = Cx  Est with no control input: zdot = Fz + Ky, xhat = z + Hy
% sysEst = ss(F,[T*B,K],eye(nx),[zeros(size(T*B)),H]); %

%% Calculate discrete forms of A,B
A2 = F*F;
A3 = F*A2;
Apre = (1.0/24.0)*DT^4*A3+(1.0/6.0)*DT^3*A2+0.5*DT^2*F+DT*eye(size(F));

%% Finish calculation of A,B
Ak = Apre*F + eye(size(F));
Bk = Apre*[T*B,K];
Ck = eye(size(F));
Dk = [zeros(size(T*B)),H];

== matlab function test_SimulinkMdl2_qLPVMPCbeta_UIO_testOL/MATLAB Function ==
  settings: updateMethod=DISCRETE
  data: rhoP input; lambda input; beta input; Cq input; A output; Bout output; DT input
function [A,Bout] = ABqL_WT_beta_m(rhoP,lambda,beta,Cq,DT)
% ABqL calculates system (A) and input (B) matrix for quasiLPV
% representation for ve
%
% Inputs: * Ts: Sampling time
%         * AwithV: Scheduling parameter vector: AwithV = V
%
% Outputs: * A: System matrix A(AwithV) at current estimated air speed AwithV, discretised with Ts
%          * B: Input matrix B(AwithV) at current AwithV, discretised with Ts

% Pablo S.G. Cisneros, Herbert Werner, ICS TUHH
% modified for WECS simulation: Antje Dittmer

persistent lambdaVec pitchVec CqVec Cqdlambda Cqdbeta

if isempty(lambdaVec)
    lambdaVec =  lambda;
    pitchVec = beta;
    CqVec = Cq;
    %% Compute gradients %%[Cpdlambda,Cpdbeta] = gradient(Cp,mean(diff(Xq(1,:))),mean(diff(Yq(:,1))));
    [Cqdlambda,Cqdbeta] = gradient(CqVec,mean(diff(lambda)),mean(diff(beta))); %dcQ/dbetaDeg * dbetaDeg/dbetaRad *betaRAd
end

%% Parameters
if length(rhoP) == 1
    Vbar = rhoP; % Vbar
    LUT_V = 4:25; % LUT table rows
    
    LUT_omega = ...%[0.4815, 0.6017,0.7217,0.8413,0.9603,1.0786,1.1949, repmat(1.2671,1,15)];
        [0.7458832277625318 0.77759738173519954 0.820732502042672 ...
        0.87379091011167287 0.93538972625666472 1.0429417531956238 ...
        1.1591854391157337 1.2371015764176956 1.2554479267196832 ...
        1.2547857982936621 1.2545286368009017 1.2546177195393646 ...
        1.2545376249695805 1.2545426663335242 1.2545426663335242 ...
        1.2545426663335242 1.2545426663335242 1.2545426663335242 ...
        1.2545426663335242 1.2545426663335242 1.2545426663335242 ...
        1.2545426663335242];
    
    LUT_beta =  [0 0 0 0 0 0 0 0 0.064193209888351435 0.11259119004615419 ...
        0.14929546421559495 0.18081611050661253 0.20926497731412011 ...
        0.23701571242082992 0.26197392072434883 0.28536133270107289 ...
        0.30770154712660031 0.32934362985133 0.35028758087526196 ...
        0.37035886727319672 0.38973202197033374 0.40858157789187255 ...
        ];
    
    
    % Get omegabar and beta
    omegabar = interp1(LUT_V,LUT_omega,Vbar,'pchip');
    beta_bar = interp1(LUT_V,LUT_beta,Vbar,'pchip');
    
elseif length(rhoP) == 3
    % rho = xdotk_1([1,3,4]); % Tg not included: [Omega [1/s], beta[rad], V [m/s]];
    Vbar = rhoP(3);
    omegabar = rhoP(1); % pass OmegaR OmegaG/Ng as approximation of omegaR
    beta_bar = rhoP(2);
    
else
    error('Unexpected length of scheduling parameter rho')
end

%% Physical and model constants
rho = 1.2250;
rb = 63; % m blade radius
Ng = 97; %Gearbox ratio
Jr = (115926 + 3 * 11.776e6) *1; %kg*m^2 Inertia of the rotor (Hub inertia + 3 blades
Jg = 534.116;% * Ng^2; %kg*m^2 Inertia of the generator (HSS)
Jgr = Jg * Ng^2; % Inertia of the generator in LSS
Ks = 867637000; %Nm/rad Stiffness of the transmission
Bs = 6215000;  %Nm/rad/sec        %Damping of the transmission
tau_g = 0.01; % for pitch actuator and airspeed

%% Lambda
Lambda_bar = omegabar*rb/Vbar;
dlambdadomega= rb/Vbar;
dlambdadV = - omegabar*rb/Vbar^2;

%% Grid points
Cqb = interp2(lambdaVec,pitchVec,Cq,Lambda_bar,beta_bar);
dCqdlambdab = interp2(lambdaVec,pitchVec,Cqdlambda,Lambda_bar,beta_bar);
dCqdbetab = interp2(lambdaVec,pitchVec,Cqdbeta,Lambda_bar,beta_bar);
%% Tr=0.5*pi*rb^3*Cq*v^2
dTrdomega = 0.5*rho*pi*rb^3*(dCqdlambdab*dlambdadomega)*Vbar^2;% br = dTr/domega
dTrdbeta = 0.5*rho*pi*rb^3*dCqdbetab*Vbar^2;% Krb = dTr/dbeta
dTrdV =  2*0.5*rho*pi*rb^3*Vbar*Cqb + ...
    0.5*rho*pi*rb^3*Vbar^2*dCqdlambdab*dlambdadV;

%% Create system matrix A:
% States: [Theta_s [rad], omega_r [rad/s], omega_gr [rad/s], T_g [Nm]]
% States for model xA = [y, xdot] with y = [Tg, beta]
% x = [ThetaS, OmegaR, OmegaG, Tg, beta,]
Atemp = [[0,1,-1,0] ;
    [-Ks/Jr, (-Bs + dTrdomega)/Jr, Bs/Jr,0];
    Ks/Jgr, Bs/Jgr, -Bs/Jgr, -Ng/Jgr;
    zeros(1,3), -1/tau_g];

%% Create input matrix B
% Input orig model: V [m/s], T_g_ref [Nm], beta [rad],
% -> vel model: Vdot [m/s^2]  , T_g_refDot [Nm/s]
% for beta: Vdot [m/s^2]  T_g_refDot [Nm/s] betaDot [rad/s],
Btemp = [zeros(1,3); dTrdV/Jr, 0 dTrdbeta/Jr; zeros(1,3);  0,  1/tau_g,0];

% With Beta
Aeval = [Atemp,Btemp(:,3); zeros(1, size(Atemp,2)), -1/tau_g];
Beval = [Btemp; zeros(1, size(Btemp,2))];
Beval(:,3) = 0;
Beval(end,3) = 1/tau_g;


%% Check rank
Bu = Beval(:,2:3);
Bd = Beval(:,1);
nxEval = size(Aeval,2);

% Also create an additional state for the disturbance
tau1 =  1/DT *0.1;
A =[[Aeval, zeros(nxEval,1)]; [zeros(1,nxEval),-tau1]];
E = [Bd;tau1]; %xd_dot = -xd + Ed
B = [Bu; zeros(1,2)];
Bout = [E,B];
%fprintf('rank(C*E) is %d; rank(E) is %d\n', rank(C1*E1),rank(E1));


%% Calculate observer matrices
% Ceval = [zeros(nxEval-1,1),eye(nxEval-1)]; %
% nyEval = size(Ceval,1);

%C = [Ceval, zeros(nyEval,1)]; %[zeros(1,nx),1]];
% H = E*inv((C*E)'*(C*E))*(C*E)'; %#ok<MINV,*NOPTS> display output, inv is fast enough
% nx = size(A,1);
% T = eye(nx)-H*C;
% A1 = T*A;

% Pole placement with Q and R
% Qe = eye(nxEval); %B*B'; %
% Re = C*C';
% K1 = lqr(A',C',Qe,Re)';
%
% % Calculate F and K
% F = A1 - K1*C; %T*A -K1*C
% K = K1 + F*H;
% T = eye(size(H*C)) - H*C;

% Sys with no ctrl input: xdot = Ax + Ed, y = Cx
% nd = size(E,2); %nu = 0;
%sys = ss(A,[E,B],C,zeros(ny,nd+2));

end

== matlab function test_SimulinkMdl2_qLPVMPCbeta_UIO_testOL/MATLAB Function2 ==
  settings: updateMethod=DISCRETE
  data: DT input; rhoP input; Av output; Rotor_Lambda input; Rotor_Pitch input; Rotor_cQ input; Bv output
function [Av,Bv] = ABqLd_WT(DT,rhoP,Rotor_Lambda,Rotor_Pitch,Rotor_cQ)
% ABqLd calculates system (A) and input (B) matrix for quasiLPV
% representation from ABgL and augments the states with integrating
% disturbances.
%
% Inputs: * DT: Sampling time
%         * rho: Scheduling parameter vector: rho = V
%
% Outputs: * A: Augmented system matrix A(rho) at current rho
%          * B: Augmented Input matrix B(rho) at current rho

% Pablo S.G. Cisneros, Herbert Werner, ICS TUHH

[Arho,Brho] = ABqL_WT(rhoP,Rotor_Lambda,Rotor_Pitch,Rotor_cQ);
%[Arho,Brho] = ABqL_WT_beta(rhoP,Rotor_Lambda,Rotor_Pitch,Rotor_cQ);
%[Arho, Brho, ~, ~, dTrdomega, Tr, dTrdV] = ABqL_WT_KMC(rhoP,Rotor_Lambda,Rotor_Pitch,Rotor_cQ);

%% Calculate discrete forms of A,B
A2 = Arho*Arho;
A3 = Arho*A2;
Apre = (1.0/24.0)*DT^4*A3+(1.0/6.0)*DT^3*A2+0.5*DT^2*Arho+DT*eye(size(Arho));

%% Finish calculation of A,B
Ak = Apre*Arho + eye(size(Arho));
Bk = Apre*Brho;

%% Calculate new matrices augmented system
ny = 2; %
nx = size(Arho,1);
nyvec = nx-1:nx; % 
nd = 1;% B: columns disturbance input
nuvec = 2:3; % B: columns control input
Cdiag = diag([97,1]); %eye(ny); %diag([97,1]);

A = [eye(2) Cdiag* Ak(3:4,:);
    zeros(size(Ak,1),ny), Ak];

B = [Cdiag* Bk(3:4,2:3); Bk(:,2:3)];
Bv1 = [Cdiag* Bk(3:4,1); Bk(:,1)];

Av = [A,Bv1; [zeros(nd,(nx+ny)) 0 *eye(nd)]];
Bv = [B; zeros(nd, size(B,2))];


end

== matlab function test_SimulinkMdl2_qLPVMPCbeta_UIO_testOL/MATLAB Function3 ==
  settings: updateMethod=DISCRETE
  data: rhoP input; pitch input; torque input; lambda input; beta input; Cq input; Tr output; Ft output; DT input
function [Tr,Ft] = getTrFt(rhoP,pitch,torque,lambda,beta,Cq,DT)
% getTrFt
% representation for ve
%
% Inputs: * Ts: Sampling time
%         * AwithV: Scheduling parameter vector: AwithV = V
%
% Outputs: * A: System matrix A(AwithV) at current estimated air speed AwithV, discretised with Ts
%          * B: Input matrix B(AwithV) at current AwithV, discretised with Ts

% Pablo S.G. Cisneros, Herbert Werner, ICS TUHH
% modified for WECS simulation: Antje Dittmer

persistent lambdaVec pitchVec CqVec Cqdlambda Cqdbeta

if isempty(lambdaVec)
    lambdaVec =  lambda;
    pitchVec = beta;
    CqVec = Cq;
    %% Compute gradients %%[Cpdlambda,Cpdbeta] = gradient(Cp,mean(diff(Xq(1,:))),mean(diff(Yq(:,1))));
    %[Cqdlambda,Cqdbeta] = gradient(CqVec,mean(diff(lambda)),mean(diff(beta))); %dcQ/dbetaDeg * dbetaDeg/dbetaRad *betaRAd
end

%% Physical and model constants
rho = 1.2250;
rb = 63; % m blade radius
Ng = 97; %Gearbox ratio
Jr = (115926 + 3 * 11.776e6) *1; %kg*m^2 Inertia of the rotor (Hub inertia + 3 blades
Jg = 534.116;% * Ng^2; %kg*m^2 Inertia of the generator (HSS)
Jgr = Jg * Ng^2; % Inertia of the generator in LSS
Ks = 867637000; %Nm/rad Stiffness of the transmission
Bs = 6215000;  %Nm/rad/sec        %Damping of the transmission
tau_g = 0.01; % for pitch actuator and airspeed

%% Lambda
Lambda_bar = omegabar*rb/Vbar;
dlambdadomega= rb/Vbar;
dlambdadV = - omegabar*rb/Vbar^2;

%% Grid points
Cqb = interp2(lambdaVec,pitchVec,Cq,Lambda_bar,beta_bar);
dCqdlambdab = interp2(lambdaVec,pitchVec,Cqdlambda,Lambda_bar,beta_bar);
dCqdbetab = interp2(lambdaVec,pitchVec,Cqdbeta,Lambda_bar,beta_bar);
%% Tr=0.5*pi*rb^3*Cq*v^2
dTrdomega = 0.5*rho*pi*rb^3*(dCqdlambdab*dlambdadomega)*Vbar^2;% br = dTr/domega
dTrdbeta = 0.5*rho*pi*rb^3*dCqdbetab*Vbar^2;% Krb = dTr/dbeta
dTrdV =  2*0.5*rho*pi*rb^3*Vbar*Cqb + ...
    0.5*rho*pi*rb^3*Vbar^2*dCqdlambdab*dlambdadV;

%% Create system matrix A:
% States: [Theta_s [rad], omega_r [rad/s], omega_gr [rad/s], T_g [Nm]]
% States for model xA = [y, xdot] with y = [Tg, beta]
% x = [ThetaS, OmegaR, OmegaG, Tg, beta,]
Atemp = [[0,1,-1,0] ;
    [-Ks/Jr, (-Bs + dTrdomega)/Jr, Bs/Jr,0];
    Ks/Jgr, Bs/Jgr, -Bs/Jgr, -Ng/Jgr;
    zeros(1,3), -1/tau_g];

%% Create input matrix B
% Input orig model: V [m/s], T_g_ref [Nm], beta [rad],
% -> vel model: Vdot [m/s^2]  , T_g_refDot [Nm/s]
% for beta: Vdot [m/s^2]  T_g_refDot [Nm/s] betaDot [rad/s],
Btemp = [zeros(1,3); dTrdV/Jr, 0 dTrdbeta/Jr; zeros(1,3);  0,  1/tau_g,0];

% With Beta
Aeval = [Atemp,Btemp(:,3); zeros(1, size(Atemp,2)), -1/tau_g];
Beval = [Btemp; zeros(1, size(Btemp,2))];
Beval(:,3) = 0;
Beval(end,3) = 1/tau_g;


%% Check rank
Bu = Beval(:,2:3);
Bd = Beval(:,1);
nxEval = size(Aeval,2);

% Also create an additional state for the disturbance
tau1 =  1/DT *0.1;
A =[[Aeval, zeros(nxEval,1)]; [zeros(1,nxEval),-tau1]];
E = [Bd;tau1]; %xd_dot = -xd + Ed
B = [Bu; zeros(1,2)];
Bout = [E,B];

end

% %% Parameters
% if length(rhoP) == 1
%     Vbar = rhoP; % Vbar
%     LUT_V = 4:25; % LUT table rows
%     
%     LUT_omega = ...%[0.4815, 0.6017,0.7217,0.8413,0.9603,1.0786,1.1949, repmat(1.2671,1,15)];
%         [0.7458832277625318 0.77759738173519954 0.820732502042672 ...
%         0.87379091011167287 0.93538972625666472 1.0429417531956238 ...
%         1.1591854391157337 1.2371015764176956 1.2554479267196832 ...
%         1.2547857982936621 1.2545286368009017 1.2546177195393646 ...
%         1.2545376249695805 1.2545426663335242 1.2545426663335242 ...
%         1.2545426663335242 1.2545426663335242 1.2545426663335242 ...
%         1.2545426663335242 1.2545426663335242 1.2545426663335242 ...
%         1.2545426663335242];
%     
%     LUT_beta =  [0 0 0 0 0 0 0 0 0.064193209888351435 0.11259119004615419 ...
%         0.14929546421559495 0.18081611050661253 0.20926497731412011 ...
%         0.23701571242082992 0.26197392072434883 0.28536133270107289 ...
%         0.30770154712660031 0.32934362985133 0.35028758087526196 ...
%         0.37035886727319672 0.38973202197033374 0.40858157789187255 ...
%         ];
%     
%     
%     % Get omegabar and beta
%     omegabar = interp1(LUT_V,LUT_omega,Vbar,'pchip');
%     beta_bar = interp1(LUT_V,LUT_beta,Vbar,'pchip');
%     
% elseif length(rhoP) == 3
%     % rho = xdotk_1([1,3,4]); % Tg not included: [Omega [1/s], beta[rad], V [m/s]];
%     Vbar = rhoP(3);
%     omegabar = rhoP(1); % pass OmegaR OmegaG/Ng as approximation of omegaR
%     beta_bar = rhoP(2);
%     
% else
%     error('Unexpected length of scheduling parameter rho')
% end
